simulink model "UOTR"  (Simulink 7.1)
settings: Solver=ode15s  StartTime=0.0  StopTime=3600
settings Model: Creator=edsoncv  LastModifiedBy=HP  ExtModeTrigMode=oneshot  ExtModeArmWhenConnect=off
settings SolverCC: MaxConsecutiveMinStep=auto
settings DataIOCC: LimitDataPoints=off  SaveFormat=StructureWithTime  SaveOutput=off  SaveTime=off  TimeSaveName=t  OutputSaveName=y
settings OptimizationCC: BlockReduction=off  BooleanDataType=off
settings DebuggingCC: SaveWithParameterizedLinksMsg=none  SignalResolutionControl=TryResolveAllWithWarning  SolverPrmCheckMsg=none  MultiTaskDSMMsg=warning  MultiTaskCondExecSysMsg=none  StrictBusMsg=None
settings HardwareCC: TargetUnknown=on
settings RTWCC: IncludeERTFirstTime=on
settings GRTTargetCC: TargetFcnLib=ansi_tfl_tmw.mat

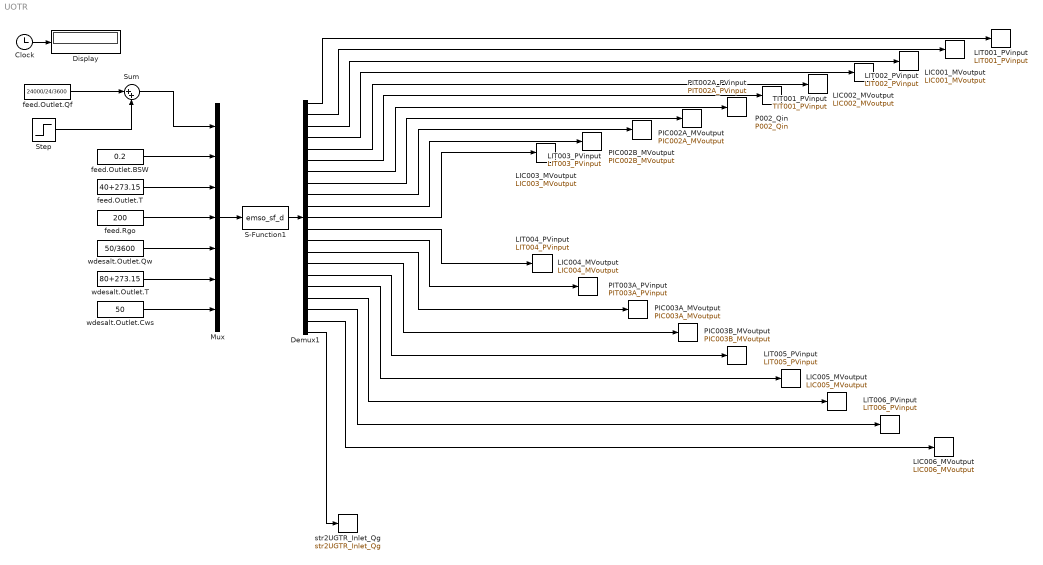
== system UOTR ==
  Clock : Clock
      settings: Decimation=10
  Demux1 : Demux  Outputs=21
  Display : Display
  LIC001_MVoutput : ToWorkspace  VariableName=LIC001_MVoutput  SampleTime=-1  SaveFormat=Structure
  LIC002_MVoutput : ToWorkspace  VariableName=LIC002_MVoutput  SampleTime=-1  SaveFormat=Structure
  LIC003_MVoutput : ToWorkspace  VariableName=LIC003_MVoutput  SampleTime=-1  SaveFormat=Structure
  LIC004_MVoutput : ToWorkspace  VariableName=LIC004_MVoutput  SampleTime=-1  SaveFormat=Structure
  LIC005_MVoutput : ToWorkspace  VariableName=LIC005_MVoutput  SampleTime=-1  SaveFormat=Structure
  LIC006_MVoutput : ToWorkspace  VariableName=LIC006_MVoutput  SampleTime=-1  SaveFormat=Structure
  LIT001_PVinput : ToWorkspace  VariableName=LIT001_PVinput  SampleTime=-1  SaveFormat=Structure
  LIT002_PVinput : ToWorkspace  VariableName=LIT002_PVinput  SampleTime=-1  SaveFormat=Structure
  LIT003_PVinput : ToWorkspace  VariableName=LIT003_PVinput  SampleTime=-1  SaveFormat=Structure
  LIT004_PVinput : ToWorkspace  VariableName=LIT004_PVinput  SampleTime=-1  SaveFormat=Structure
  LIT005_PVinput : ToWorkspace  VariableName=LIT005_PVinput  SampleTime=-1  SaveFormat=Structure
  LIT006_PVinput : ToWorkspace  VariableName=LIT006_PVinput  SampleTime=-1  SaveFormat=Structure
  Mux : Mux  Inputs=7
  P002_Qin : ToWorkspace  VariableName=P002_Qin  SampleTime=-1  SaveFormat=Structure
  PIC002A_MVoutput : ToWorkspace  VariableName=PIC002A_MVoutput  SampleTime=-1  SaveFormat=Structure
  PIC002B_MVoutput : ToWorkspace  VariableName=PIC002B_MVoutput  SampleTime=-1  SaveFormat=Structure
  PIC003A_MVoutput : ToWorkspace  VariableName=PIC003A_MVoutput  SampleTime=-1  SaveFormat=Structure
  PIC003B_MVoutput : ToWorkspace  VariableName=PIC003B_MVoutput  SampleTime=-1  SaveFormat=Structure
  PIT002A_PVinput : ToWorkspace  VariableName=PIT002A_PVinput  SampleTime=-1  SaveFormat=Structure
  PIT003A_PVinput : ToWorkspace  VariableName=PIT003A_PVinput  SampleTime=-1  SaveFormat=Structure
  S-Function1 : S-Function  FunctionName=emso_sf_d  Parameters='UOTR.ems',7,21,1  EnableBusSupport=off
  Step : Step  Time=300  After=-2000/24/3600  SampleTime=0
  Sum : Sum  Inputs=|++  OutDataType=sfix(16)  OutScaling=2^0
  TIT001_PVinput : ToWorkspace  VariableName=TIT001_PVinput  SampleTime=-1  SaveFormat=Structure
  feed.Outlet.BSW : Constant  Value=0.2  OutDataType=sfix(16)  OutScaling=2^0
  feed.Outlet.Qf : Constant  Value=24000/24/3600  OutDataType=sfix(16)  OutScaling=2^0
  feed.Outlet.T : Constant  Value=40+273.15  OutDataType=sfix(16)  OutScaling=2^0
  feed.Rgo : Constant  Value=200  OutDataType=sfix(16)  OutScaling=2^0
  str2UGTR_Inlet_Qg : ToWorkspace  VariableName=str2UGTR_Inlet_Qg  SampleTime=-1  SaveFormat=Structure
  wdesalt.Outlet.Cws : Constant  Value=50  OutDataType=sfix(16)  OutScaling=2^0
  wdesalt.Outlet.Qw : Constant  Value=50/3600  OutDataType=sfix(16)  OutScaling=2^0
  wdesalt.Outlet.T : Constant  Value=80+273.15  OutDataType=sfix(16)  OutScaling=2^0
  wires:
  Clock/1 -> Display/1
  S-Function1/1 -> Demux1/1
  Mux/1 -> S-Function1/1
  feed.Outlet.Qf/1 -> Sum/1
  wdesalt.Outlet.Cws/1 -> Mux/7
  wdesalt.Outlet.T/1 -> Mux/6
  wdesalt.Outlet.Qw/1 -> Mux/5
  feed.Rgo/1 -> Mux/4
  feed.Outlet.T/1 -> Mux/3
  feed.Outlet.BSW/1 -> Mux/2
  Demux1/1 -> LIT001_PVinput/1
  Demux1/2 -> LIC001_MVoutput/1
  Demux1/3 -> LIT002_PVinput/1
  Demux1/4 -> LIC002_MVoutput/1
  Demux1/5 -> TIT001_PVinput/1
  Demux1/6 -> P002_Qin/1
  Demux1/7 -> PIT002A_PVinput/1
  Demux1/8 -> PIC002A_MVoutput/1
  Demux1/9 -> PIC002B_MVoutput/1
  Demux1/10 -> LIT003_PVinput/1
  Demux1/11 -> LIC003_MVoutput/1
  Demux1/12 -> LIT004_PVinput/1
  Demux1/13 -> LIC004_MVoutput/1
  Demux1/14 -> PIT003A_PVinput/1
  Demux1/15 -> PIC003A_MVoutput/1
  Demux1/16 -> PIC003B_MVoutput/1
  Demux1/17 -> LIT005_PVinput/1
  Demux1/18 -> LIC005_MVoutput/1
  Demux1/19 -> LIT006_PVinput/1
  Demux1/20 -> LIC006_MVoutput/1
  Step/1 -> Sum/2
  Sum/1 -> Mux/1
  Demux1/21 -> str2UGTR_Inlet_Qg/1
